simulink library "casper_library_misc"  (R2021a)
settings: Solver=ode45  StartTime=0.0  StopTime=10.0  RelTol=1e-3
libraries: xbsIndex_r4 x168, $bdroot x11, xps_library x6, simulink x4
(part 1 of 3)
settings Model: Creator=mdexter  LastModifiedBy=mcb
settings SolverCC: AlgebraicLoopSolver=TrustRegion
settings DataIOCC: LimitDataPoints=on  SaveFormat=Array  SignalLoggingSaveFormat=ModelDataLogs  ReturnWorkspaceOutputs=off
settings OptimizationCC: BlockReduction=off  BooleanDataType=off  ExpressionDepthLimit=2147483647  LifeSpan=inf
settings DebuggingCC: SaveWithParameterizedLinksMsg=none  UnderspecifiedInitializationDetection=Classic  MergeDetectMultiDrivingBlocksExec=none  SignalResolutionControl=TryResolveAllWithWarning  FcnCallInpInsideContextMsg=warning  AllowSymbolicDim=off  StateNameClashWarn=warning  SFUnexpectedBacktrackingDiag=warning  SFNoUnconditionalDefaultTransitionDiag=warning  SFExecutionAtInitializationDiag=none  SFMachineParentedDataDiag=warning  ArithmeticOperatorsInVariantConditions=warning
settings HardwareCC: ProdBitPerPointer=32  ProdBitPerSizeT=32  ProdBitPerPtrDiffT=32  ProdLargestAtomicFloat=None  ProdIntDivRoundTo=Undefined  ProdEndianess=Unspecified  ProdWordSize=32  ProdHWDeviceType=32-bit Generic  TargetUnknown=on
settings ModelReferenceCC: PropagateSignalLabelsOutOfModel=off
settings SFSimCC: SimUseLocalCustomCode=off  CustomCodeUndefinedFunction=UseInterfaceOnly
settings RTWCC: RTWUseLocalCustomCode=off
settings CodeAppCC: StateflowObjectComments=on
settings GRTTargetCC: TargetLangStandard=C89/C90 (ANSI)  CombineOutputUpdateFcns=off  GRTInterface=on
settings ConfigComp: CovMetricSettings=dw  CovSaveCumulativeToWorkspaceVar=on  CovSaveSingleToWorkspaceVar=on  CovExternalEMLEnable=off

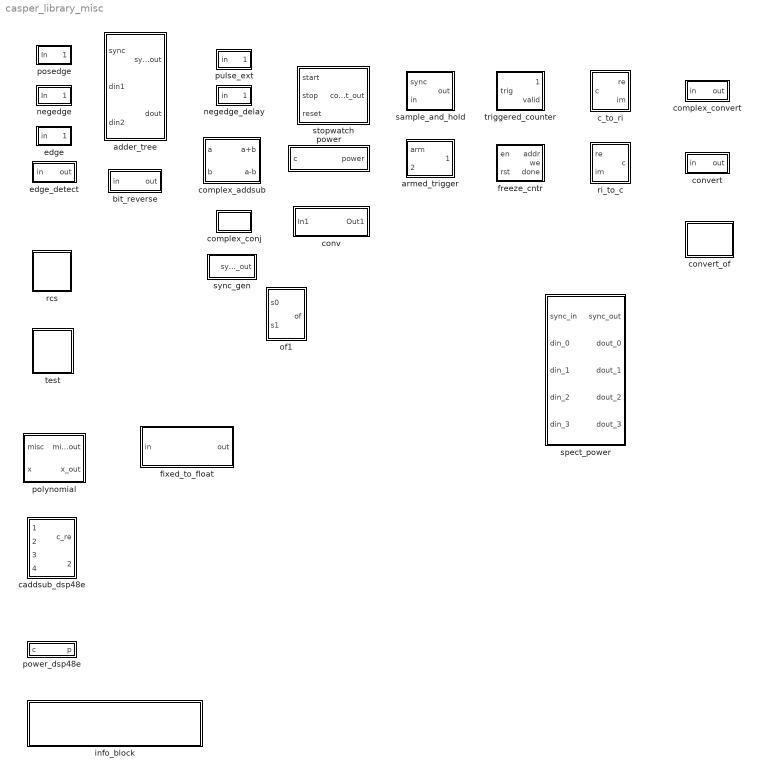
== system casper_library_misc ==
  adder_tree : Subsystem  mask(adder_tree){n_inputs=2, csp_latency=1, adder_imp=Fabric, first_stage_hdl=on, floating_point=off, dvalid_en=off, float_type=single, frac_width=0, exp_width=0}
      mask prompts: n_inputs "Number of Inputs"; csp_latency "Add Latency"; adder_imp "Adder implementation"; first_stage_hdl "Use behavioural HDL for first stage of adders"; floating_point "floating point"; float_type "float type"; frac_width "fraction length"; exp_width "exponent length"
      mask help:
      | Sums all inputs using a tree of adds and delays.
      |
      | Number of inputs: The number of inputs to the block to be summed
      | Add latency: The number of clock cycles to perform one addition (affects timing)..
      | Adder implementation: choice of fabric or DSP48E core, or behavioral HDL
      | Use behavioural HDL for first stage of adders: Causes the first stage of adders to be absorbed into DSP blocks if multipliers precede them (Virtex 5). Overrides Adder implementation
      mask init:
      | adder_tree_init(gcb, ...
      |     'n_inputs', n_inputs, ...
      |     'csp_latency', csp_latency, ...
      |     'adder_imp', adder_imp, ...
      |     'dvalid_en', dvalid_en, ...
      |     'floating_point', floating_point, ...
      |     'float_type', float_type, ...
      |     'exp_width', exp_width, ...
      |     'frac_width', frac_width, ...     
      |     'first_stage_hdl', first_stage_hdl);
      settings: AttributesFormatString=latency 1
      mask Help: eval('xlWeb(''http://casper.berkeley.edu/wiki/Adder_tree'')')
      mask TypeOptions adder_imp: Behavioral | Fabric | DSP48
      mask Callback floating_point:
      | onoff = get_param(gcb, 'floating_point');
      | if strcmp(onoff,'on')
      |     enable_fixpt = 'off';
      |     set_param_state(gcb, 'float_type', 'on')
      | 
      |     f_type = get_param(gcb, 'float_type');
      |     if strcmp(f_type,'custom')
      |         set_param_state(gcb, 'exp_width', 'on')
      |         set_param_state(gcb, 'frac_width', 'on')
      |     else
      |         set_param_state(gcb, 'exp_width', 'off')
      |         set_param_state(gcb, 'frac_width', 'off')
      |     end
      | 
      | 
      | else
      |     enable_fixpt = 'on';
      |     set_param_state(gcb, 'float_type', 'off')
      |     set_param_state(gcb, 'exp_width', 'off')
      |     set_param_state(gcb, 'frac_width', 'off')
      | end
      mask TypeOptions float_type: single | custom
      mask Callback float_type:
      | f_type = get_param(gcb, 'float_type');
      | if strcmp(f_type,'custom')
      |     set_param_state(gcb, 'exp_width', 'on')
      |     set_param_state(gcb, 'frac_width', 'on')
      | else
      |     set_param_state(gcb, 'exp_width', 'off')
      |     set_param_state(gcb, 'frac_width', 'off')
      | end
  armed_trigger : Subsystem  mask(Armed Trigger){}
      mask help: Makes a boolean trigger signal armable.
      mask Help: The trig_out port will go high for one cycle during the first high cycle of trig_in.  Thereafter, trig_out will only go high for one cycle during the first high cycle of trig_in after each rising edge of arm.
  bit_reverse : Subsystem  mask(bit_reverse){n_bits=1}
      mask prompts: n_bits "Number of Bits"
      mask help: Reverses the bit order of the input. Input must be unsigned with binary point at position 0. Costs nothing in hardware.
      mask init:
      | bit_reverse_init(gcb,'n_bits', n_bits);
      settings: AttributesFormatString=1 bits
      mask Help: eval('xlWeb(''http://casper.berkeley.edu/wiki/Bit_reverse'')')
  c_to_ri : Subsystem  mask(c_to_ri){n_bits=8, bin_pt=7}
      mask prompts: n_bits "Bit Width"; bin_pt "Binary Point"
      mask help:
      | Outputs real and imaginary components of a complex input.
      | Useful for simplifying interconnects.
      | See also: Real-Imag to Complex (ri_to_c)
      mask init:
      | annotation=sprintf('%d_%d r/i',n_bits,bin_pt);
      | set_param(gcb,'AttributesFormatString',annotation);
      settings: AttributesFormatString=8_7 r/i
      mask Help: eval('xlWeb(''http://casper.berkeley.edu/wiki/C_to_ri'')')
  caddsub_dsp48e : Subsystem  mask(caddsub_dsp48e){mode=Addition, n_bits_a=18, bin_pt_a=17, n_bits_b=8, bin_pt_b=7, full_precision=on, n_bits_c=19, bin_pt_c=17, quantization=Truncate, overflow=Wrap, cast_latency=0}
      mask prompts: mode "Operation:"; n_bits_a "Bit width 'a':"; bin_pt_a "Binary point 'a':"; n_bits_b "Bit width 'b':"; bin_pt_b "Binary point 'b':"; full_precision "Full precision"; n_bits_c "Bit width out:"; bin_pt_c "Binary point out:"; cast_latency "Cast Latency:"
      mask help:
      | Adds or subtracts two complex numbers using a DSP48E.
      |
      | The two inputs can have different bit widths and binary points, but their sum cannot exceed 24 bits.
      mask init:
      | caddsub_dsp48e_init(gcb, ...
      |     'mode', mode, ...
      |     'n_bits_a', n_bits_a, ...
      |     'bin_pt_a', bin_pt_a, ...
      |     'n_bits_b', n_bits_b, ...
      |     'bin_pt_b', bin_pt_b, ...
      |     'full_precision', full_precision, ...
      |     'n_bits_c', n_bits_c, ...
      |     'bin_pt_c', bin_pt_c, ...
      |     'quantization', quantization, ...
      |     'overflow', overflow, ...
      |     'cast_latency', cast_latency);
      settings: AttributesFormatString=|
      | 18_17 + 8_7 ==> 19_17
      | Mode=Addition
      | Latency=2
      mask TypeOptions mode: Addition | Subtraction
      mask Callback full_precision:
      | thisVariable = 'full_precision';
      | affectedVars = { ...
      |     'n_bits_c', ...
      |     'bin_pt_c', ...
      |     'quantization', ...
      |     'overflow', ...
      |     'cast_latency', ...
      | };
      | 
      | thisBlock = gcb();
      | thisVarState = get_param(thisBlock, thisVariable);
      | maskNames = get_param(thisBlock, 'MaskNames');
      | maskEnables = get_param(thisBlock, 'MaskEnables');
      | 
      | if strcmp(thisVarState, 'on'),
      |     targVarState = 'off';
      | else,
      |     targVarState = 'on';
      | end
      | 
      | for varName = affectedVars
      |     varIndex = find(ismember(maskNames, varName));
      |     maskEnables{varIndex} = targVarState;
      | end
      | 
      | set_param(thisBlock, 'MaskEnables', maskEnables);
      mask TypeOptions quantization: Truncate | Round  (unbiased: +/- Inf) | Round  (unbiased: Even Values)
      mask TypeOptions overflow: Wrap | Saturate | Flag as error
  complex_addsub : Subsystem  mask(complex_addsub){BitWidth=18, add_latency=2}
      mask prompts: BitWidth "Bit Wdith"; add_latency "Add Latency"
      mask help:
      | Adds and subtracts the complex inputs.
      | If a = w + ix, b = y + iz then
      | a+b = (w+y)/2 + i(x-z)/2 and
      | a-b = (x+z)/2 + i(y-w)/2
  complex_conj : Subsystem  mask(complex_conj){n_inputs=0, n_bits=18, bin_pt=17, csp_latency=1, overflow=Wrap, floating_point=on, float_type=single, exp_width=8, frac_width=24}
      mask prompts: n_inputs "number simultaneous inputs"; n_bits "input bitwidth"; bin_pt "input binary point"; csp_latency "latency"; overflow "overflow strategy"; floating_point "floating point"; exp_width "exponent width"; frac_width "fraction width"
      mask help: Finds the complex conjugate of complex inputs.
      mask init:
      | complex_conj_init(gcb, ...
      |     'n_inputs', n_inputs, ...
      |     'n_bits', n_bits, ...
      |     'bin_pt', bin_pt, ...
      |     'floating_point', floating_point, ...
      |     'float_type', float_type, ...
      |     'exp_width', exp_width, ...
      |     'frac_width', frac_width, ...        
      |     'csp_latency', csp_latency, ...
      |     'overflow', overflow);
      mask TypeOptions overflow: Wrap | Saturate | Flag as error
      mask Callback floating_point:
      | onoff = get_param(gcb, 'floating_point');
      | if strcmp(onoff,'on')
      |     enable_fixpt = 'off'
      |     set_param_state(gcb, 'float_type', 'on')
      | 
      |     f_type = get_param(gcb, 'float_type')
      |     if strcmp(f_type,'custom')
      |         set_param_state(gcb, 'exp_width', 'on')
      |         set_param_state(gcb, 'frac_width', 'on')
      |     else
      |         set_param_state(gcb, 'exp_width', 'off')
      |         set_param_state(gcb, 'frac_width', 'off')
      |     end
      | 
      | 
      | else
      |     enable_fixpt = 'on'
      |     set_param_state(gcb, 'float_type', 'off')
      |     set_param_state(gcb, 'exp_width', 'off')
      |     set_param_state(gcb, 'frac_width', 'off')
      | end
      | 
      | set_param_state(gcb, 'n_bits', enable_fixpt)
      | set_param_state(gcb, 'bin_pt', enable_fixpt)
      mask TypeOptions float_type: single | custom
      mask Callback float_type:
      | f_type = get_param(gcb, 'float_type')
      | if strcmp(f_type,'custom')
      |     set_param_state(gcb, 'exp_width', 'on')
      |     set_param_state(gcb, 'frac_width', 'on')
      | else
      |     set_param_state(gcb, 'exp_width', 'off')
      |     set_param_state(gcb, 'frac_width', 'off')
      | end
  complex_convert : Subsystem  mask(complex_convert){n_bits_in=8, bin_pt_in=7, n_bits_out=8, bin_pt_out=7, quantization=Truncate, overflow=Wrap, csp_latency=3}
      mask prompts: n_bits_in "Bit Width In"; bin_pt_in "Binary Point In"; n_bits_out "Bit Width Out"; bin_pt_out "Binary Point Out"; csp_latency "Latency"
      mask help: Convert real and imaginary components of a complex input to the specified bit width and precision.
      mask init:
      | complex_convert_init(gcb, ...
      |     'n_bits_in',n_bits_in,...
      |     'bin_pt_in',bin_pt_in, ...
      |     'n_bits_out',n_bits_out,...
      |     'bin_pt_out',bin_pt_out,...
      |     'quantization',quantization,...
      |     'overflow',overflow,...
      |     'latency',csp_latency);
      settings: AttributesFormatString=|
      | 8_7 ==> 8_7
      | truncate, wrap
      | latency = 3
      mask Help:
      | <pre>
      | Description::
      | 
      | Outputs (complex) converted version of the (complex) input.
      | 
      | Mask Parameters::
      | 
      | Bit Width In (n_bits_in): Specifies the width of the real/imaginary input components.
      | Assumed equal for both components.
      | 
      | Binary Point In (bin_pt_in): Specifies the binary point location in the real/imag input components.
      | Assumed equal for both components.
      | 
      | Bit Width Out (n_bits_out): Specifies the width of the real/imaginary output components.
      | Assumed equal for both components.
      | 
      | Binary Point Out (bin_pt_out): Specifies the binary point location in the real/imag output components.
      | Assumed equal for both components.
      | 
      | Quantization (quantization): Specifies quantization handling.
      | 
      | Overflow (overflow): Specifies overflow handling.
      | 
      | Latency (latency): Specifies the latency of the underlying convert blocks, which is the overall
      | latency of this block as well.
      | </pre>
      mask TypeOptions quantization: Truncate | Round  (unbiased: +/- Inf) | Round  (unbiased: Even Values)
      mask TypeOptions overflow: Wrap | Saturate | Error
  conv : Subsystem
      mask help:
      | Converts an (8-bit) unsigned number to 2's complement.
      | This block should eventually be able to handle arbitrary
      | width inputs.
  convert : Subsystem  mask(convert){bin_pt_in=7, n_bits_out=4, bin_pt_out=3, quantization=Truncate, overflow=Wrap, csp_latency=4, implementation=0}
      mask prompts: bin_pt_in "Binary Point In"; n_bits_out "Bit Width Out"; bin_pt_out "Binary Point Out"; csp_latency "Latency"; implementation "Implementation (0=Fabric Core, 1=DSP Core, 2=Behavioural)"
      mask help:
      | Convert input value to the specified bit width and precision.
      |
      | Does not support upscaling number of fractional bits (eg 8_5 to 8_4 is ok, but not 8_4 to 8_5).
      mask init:
      | convert_init(gcb, ...
      |     'bin_pt_in',bin_pt_in, ...
      |     'n_bits_out',n_bits_out,...
      |     'bin_pt_out',bin_pt_out, ...
      |     'quantization',quantization,...
      |     'overflow',overflow,...
      |     'csp_latency',csp_latency,...
      |     'implementation', implementation);
      settings: AttributesFormatString=|
      | N_7 ==> 4_3
      | truncate, wrap
      | latency = 4
      mask Help:
      | <pre>
      | Description::
      | 
      | Outputs converted version of the input.
      | 
      | Mask Parameters::
      | 
      | Binary Point In (bin_pt_in): Specifies the binary point location in the input.
      | 
      | Bit Width Out (n_bits_out): Specifies the width of the output.
      | 
      | Binary Point Out (bin_pt_out): Specifies the binary point location in the output.
      | 
      | Quantization (quantization): Specifies quantization handling.
      | 
      | Overflow (overflow): Specifies overflow handling.
      | 
      | Latency (latency): Specifies the latency of the underlying adder block, which is the overall
      | latency of this block as well.
      | </pre>
      mask TypeOptions quantization: Truncate | Round  (unbiased: +/- Inf) | Round  (unbiased: Even Values) | Round  (unbiased: Zero) | Round  (unbiased: Odd Values) | Round  (biased: Up) | Round  (biased: Down)
      mask TypeOptions overflow: Wrap | Saturate | Error
  convert_of : Subsystem  mask(convert_of){bit_width_i=0, binary_point_i=2, bit_width_o=8, binary_point_o=7, csp_latency=2, overflow=Wrap, quantization=Truncate}
      mask prompts: bit_width_i "Bit Width In"; binary_point_i "Binary Point In"; bit_width_o "Bit Width Out"; binary_point_o "Binary Point Out"; csp_latency "Latency"; overflow "Overflow Behaviour"; quantization "Quantization Behaviour"
      mask help:
      | Converts from one 2's complement bit-width
      | and/or binary point position to another.
      | Includes underflow/overflow indicator.
      mask init:
      | convert_of_init(gcb, ...
      |     'bit_width_i', bit_width_i, ...
      |     'binary_point_i', binary_point_i, ...
      |     'bit_width_o', bit_width_o, ...
      |     'binary_point_o', binary_point_o, ...
      |     'latency',csp_latency, ...
      |     'overflow', overflow, ...
      |     'quantization', quantization);
      mask TypeOptions overflow: Wrap | Saturate | Error
      mask TypeOptions quantization: Truncate | Round  (unbiased: +/- Inf) | Round  (unbiased: even values)
  edge : Subsystem  mask(edge){}
      mask help: Outputs true if a boolean input signal is not equal to its value last clock.
      mask init:
      | deprecation_warning('the edge block is to be removed from the casper library, please use the edge_detect block instead', 'edge');
      settings: CopyFcn=deprecation_warning('the edge block is to be removed from the casper library, please use the edge_detect block instead','edge')
      mask Help: eval('xlWeb(''http://casper.berkeley.edu/wiki/Edge'')')
  edge_detect : Subsystem  mask(edge_detect){edge=Rising, polarity=Active High, x_in=[0 0.08 0.08 0.16 0.16 0.24 0.24 0.32 0.32 0.4], y_in=[-1 -1  1  1  1  1  1  1  1  1], x_out=[0.6 0.68 0.68 0.76 0.76 0.84 0.84 0.92 0.92 1], y_out=[-1 -1  1  1 -1 -1 -1 -1 -1 -1]}
      mask prompts: edge "Edge Type"; polarity "Output Polarity"; x_in "Input X Positions"; y_in "Input Y Positions"; x_out "Output X Positions"; y_out "Output Y Positions"
      mask help: Output is active for one-cycle after each edge of the specified type (i.e. rising, falling or both).
      mask init:
      | edge_detect_init(gcb,...
      |     'edge',edge,...
      |     'polarity',polarity,...
      |     'x_in',x_in,...
      |     'x_out',x_out,...
      |     'y_in',y_in,...
      |     'y_out',y_out);
      | 
      | x_in_num=str2num(getfield(getfield(get_param(gcb,'UserData'),'parameters'),'x_in'));
      | x_out_num=str2num(getfield(getfield(get_param(gcb,'UserData'),'parameters'),'x_out'));
      | y_in_num=str2num(getfield(getfield(get_param(gcb,'UserData'),'parameters'),'y_in'));
      | y_out_num=str2num(getfield(getfield(get_param(gcb,'UserData'),'parameters'),'y_out'));
      settings: AttributesFormatString=|
      | rising edges
      | active high
      mask Help: Output is active for one-cycle after each edge of the specified type (i.e. rising, falling, or both).  Latency is zero.
      mask TypeOptions edge: Rising | Falling | Both
      mask TypeOptions polarity: Active High | Active Low
      mask Display:
      | plot(x_in_num,0.5+y_in_num*0.2);
      | plot(x_out_num,0.5+y_out_num*0.2);
  fixed_to_float : Subsystem  mask(fixed_to_float){float_type=single, n_bits_in=18, bin_pt=17, num_vec=1, csp_latency=0}
      mask prompts: float_type "float type"; n_bits_in "input word length"; bin_pt "input binary point"; num_vec "number vectors in bus"; csp_latency "Latency"
      mask help: Convert fixed point vector (or bus of) to flaoting point
      mask TypeOptions float_type: single | custom
  freeze_cntr : Subsystem  mask(freeze_cntr){CounterBits=5}
      mask prompts: CounterBits "Counter Length (2^?)"
      mask help:
      | A freeze counter is an enabled counter which holds its final value (regardless of enables)
      | until it is reset.
      mask Help: eval('xlWeb(''http://casper.berkeley.edu/wiki/Freeze_cntr'')')
  info_block : Subsystem  Tag=casper:info  mask(comment_block){info=Any information about this system\nthat should be readable from software.\nSee documentation.}
      mask help:
      | Any comment made using this block will be parsed by the toolflow and stored in the bitstream, accessible by software.
      | It's an unevaluated string, and some characters make Matlab unhappy, so the user must define/find a data transport format if that is the intended purpose.
      settings: MoveFcn=pos = get_param(gcb, 'Position'); height = pos(4)-pos(2); txt = get_param(gcb, 'info'); set_param(gcb,'MaskValueString',txt);
      mask Display:
      | pos = get_param(gcb, 'Position');
      | height = pos(4)-pos(2);
      | txt = get_param(gcb, 'info');
      | text(10,height/2,txt);
  negedge : Subsystem  Tag=Rising Edge Detector  mask(negedge){}
      mask help: Outputs true if a boolean input signal is currently false, but was true last clock.
      mask init:
      | deprecation_warning('the negedge block is to be removed from the casper library, please use the edge_detect block instead', 'negedge');
      settings: CopyFcn=deprecation_warning('the negedge block is to be removed from the casper library, please use the edge_detect block instead','negedge')
      mask Help: eval('xlWeb(''http://casper.berkeley.edu/wiki/Negedge'')')
  negedge_delay : Subsystem  mask(negedge_delay){pulse_len=5}
      mask prompts: pulse_len "Length of Pulse"
      mask help:
      | Extends a boolean signal to be high for the specified number of clocks after
      | the last high input (negative edge).
      |
      | Minimum length is 3.
      mask init:
      | bits = ceil(log2(pulse_len+1));
      | 
      | if pulse_len < 3,
      |     errordlg('Minimum length is 3.');
      | end
  of1 : Subsystem  mask(of){bit_num=0, n_adc_bits=8}
      mask prompts: bit_num "Bit index of overflow detection bus:"; n_adc_bits "Number of bits in ADC"
      mask help: 1-cycle overflow detector for an n-bit ADC outputs (simulation only)
  polynomial : Subsystem  mask(polynomial){n_polys=0, degree=0, mult_latency=2, bits_out=18, bin_pt_out=17, conv_latency=2, quantization=Truncate, overflow=Wrap, bits_in=8, bin_pt_in=0}
      mask prompts: n_polys "Number of polynomials"; degree "Degree of polynomial"; mult_latency "Multiplier latency"; bits_out "Output number of bits"; bin_pt_out "Output binary point"; conv_latency "Convert latency"; quantization "Quantization behaviour"; overflow "Overflow behaviour"; bits_in "Bits in"; bin_pt_in "Binary point in"
      mask init:
      | polynomial_init(gcb, ...
      |     'n_polys', n_polys, ...
      |     'degree', degree, ...
      |     'mult_latency', mult_latency, ...
      |     'bits_out', bits_out, ...
      |     'bin_pt_out', bin_pt_out, ...
      |     'conv_latency', conv_latency, ...
      |     'quantization', quantization, ...
      |     'overflow', overflow, ...
      |     'bits_in', bits_in, ...
      |     'bin_pt_in', bin_pt_in);
      mask TypeOptions quantization: Truncate | Round  (unbiased: +/- Inf) | Round  (unbiased: even values)
      mask TypeOptions overflow: Wrap | Saturate | Error
  posedge : Subsystem  Tag=Rising Edge Detector  mask(posedge){}
      mask help: Outputs true if a boolean input signal is true this clock and was false last clock.
      mask init:
      | deprecation_warning('the posedge block is to be removed from the casper library, please use the edge_detect block instead', 'posedge');
      settings: CopyFcn=deprecation_warning('the posedge block is to be removed from the casper library, please use the edge_detect block instead','posedge')
      mask Help: eval('xlWeb(''http://casper.berkeley.edu/wiki/Posedge'')')
  power : Subsystem  mask(power){BitWidth=18, add_latency=2, mult_latency=3}
      mask prompts: BitWidth "Bit Width"; add_latency "Add Latency"; mult_latency "Mult Latency"
      mask help: Squares real and imaginary components of complex input and adds them.
      mask Help: eval('xlWeb(''http://casper.berkeley.edu/wiki/Power'')')
      mask Display:
      | port_label('input', 1, 'c');
      | port_label('output', 1, 'power');
      | disp(['Z^-', num2str(mult_latency+add_latency)]);
  power_dsp48e : Subsystem  mask(power_dsp48e){bitwidth=18}
      mask prompts: bitwidth "Input bit width:"
      mask help: Computes the power of a complex number using 2 DSP48Es.
      mask Display:
      | port_label('input', 1, 'c');
      | port_label('output', 1, 'p');
      | disp(['Z^-', num2str(4)]);
  pulse_ext : Subsystem  mask(pulse_ext){pulse_len=5}
      mask prompts: pulse_len "Length of Pulse"
      mask help:
      | Extends a boolean signal to be high for the specified number of clocks after
      | the last high input.
      mask init:
      | bits = ceil(log2(pulse_len+1));
      mask Help: eval('xlWeb(''http://casper.berkeley.edu/wiki/Pulse_ext'')')
  rcs : Subsystem  mask(rcs){app_src=timestamp, lib_src=timestamp, user_val=0}
      mask prompts: app_src "Application revision info to capture"; lib_src "CASPER libraries revision info to capture"; user_val "User specified value"
      mask help:
      | Embeds revision control information for the user design and libraries.
      | On failure to locate specified revision information, falls back to
      | timestamps (current time for libraries).
      | A user specified value is also stored.
      mask init:
      | rcs_init(gcb, ...
      |     'app_src', app_src, ...
      |     'lib_src', lib_src);
      mask TypeOptions app_src: timestamp | git | svn
      mask TypeOptions lib_src: timestamp | git | svn
  ri_to_c : Subsystem  mask(ri_to_c){}
      mask help:
      | Concatenates real and imaginary inputs into a complex output.
      | Useful for simplifying interconnects.
      | See also: Complex to Real-Imag (c_to_ri)
      mask Help: eval('xlWeb(''http://casper.berkeley.edu/wiki/Ri_to_c'')')
  sample_and_hold : Subsystem  mask(sample_and_hold){period=1024}
      mask prompts: period "Sample period (clocks)"
      mask help: This block will sample an input signal at a user specified rate and hold the value on the output.
  spect_power : Subsystem  mask{bitwidth=18, add_latency=2, mult_latency=3, mode=dsp48e, n_inputs=4}
      mask prompts: bitwidth "Bit Width"; add_latency "Adder Latency"; mult_latency "Mult Latency"; n_inputs "Number of Inputs"
      mask init:
      | config.source = str2func('spect_power');
      | config.depend = {'spect_power.m'};
      | config.toplevel = gcb;
      | xBlock(config, {bitwidth, add_latency, mult_latency, mode, n_inputs});
      mask TypeOptions mode: behavioral | dsp48e
  stopwatch : Subsystem  mask(stopwatch){}
      mask help: Counts the number of clocks between a start and stop pulse.
      mask Help: eval('xlWeb(''http://casper.berkeley.edu/wiki/Stopwatch'')')
  sync_gen : Subsystem  mask(sync_gen){sim_acc_len=7, fft_size=256, fft_simult_inputs=8, pfb_fir_taps=4, reorder_vec=getfield( getfield( get_param( gcb,'UserData' ), 'parameters'),'reorder_vec'), scale=1}
      mask prompts: sim_acc_len "Simulation Accumulation Length"; fft_size "FFT Size"; fft_simult_inputs "Simultaneous Inputs (FFT)"; pfb_fir_taps "Taps in pfb_fir (use 1 if no pfb_fir)"; reorder_vec "Reorder Orders (e.g. [2 2 2])"
      mask help:
      | This block computes the sync period based on system parameters as
      | described in Casper memo.  Detailed descritions of the block's
      | variables can be found in the 'Block Documentation' section of
      | the CASPER wiki.
      mask init:
      | sync_gen_init(gcb, ...
      |     'sim_acc_len', sim_acc_len, ...
      |     'fft_size', fft_size, ...
      |     'fft_simult_inputs', fft_simult_inputs,...
      |     'pfb_fir_taps', pfb_fir_taps, ...
      |     'reorder_vec', reorder_vec, ...
      |     'scale', scale);
      settings: AttributesFormatString=sim_sync_period=8960
      mask Help:
      | SyncPeriod=LCM(reorder_vec)*(acc_num)*(pfb_fir_len)*(fft_size/fft_simult_inputs)
      | 
      | See CASPER sync pulse memo for more details.
  test : Subsystem  mask(test){tests_location=/opt/casper_git_devel/casper_library/Tests, tests_file=tester_input.txt, test_type=section from block, subsection=Downconverter, block=lo_osc, stop_first_fail=on}
      mask prompts: tests_location "Location of unit tests"; tests_file "Name of test file"; test_type "Test type:"; subsection "Library subsection:"; block "Library block"; stop_first_fail "Stop testing on first failure"
      mask help: Interface to test infrastruture
      mask init:
      | test_init( gcb, ...
      |     'tests_location', tests_location, ...
      |     'tests_file', tests_file, ...
      |     'test_type', test_type, ...
      |     'subsection', subsection, ...
      |     'block', block, ...
      |     'stop_first_fail', stop_first_fail);
      mask Callback tests_file:
      | %ideally, generate sections and blocks
      | %from tests_location and test_file
      mask TypeOptions test_type: all | section | section from block | unit
  triggered_counter : Subsystem  mask{len=8}
      mask prompts: len "Run Length"

== system casper_library_misc/adder_tree ==
  sync : Inport
  din1 : Inport  Port=2
  din2 : Inport  Port=3
  addr1 : xbsIndex_r4/AddSub  mode=Addition  use_carryin=off  use_carryout=off  en=off  latency=1  precision=Full  arith_type=Unsigned  n_bits=16  bin_pt=14  quantization=Truncate  overflow=Wrap  use_behavioral_HDL=on  hw_selection=Fabric  pipelined=on  use_rpm=on  dbl_ovrd=off  block_type=addsub
  sync_delay : xbsIndex_r4/Delay  rst=off  infoeditControl=Selection of Reset will increase slice count due to use of real FFs and instead of SRLs  en=off  latency=1  reg_retiming=on  dbl_ovrd=off  block_type=delay
      settings: block_version=11.4
  sync_out : Outport  VectorParamsAs1DForOutWhenUnconnected=off
  dout : Outport  Port=2  VectorParamsAs1DForOutWhenUnconnected=off
  wires:
  sync/1 -> sync_delay/1
  sync_delay/1 -> sync_out/1
  din1/1 -> addr1/1
  din2/1 -> addr1/2
  addr1/1 -> dout/1

== system casper_library_misc/armed_trigger ==
  arm : Inport
  trig_in : Inport  Port=2
  Constant2 : xbsIndex_r4/Constant  const=0  gui_display_data_type=Fixed-point  arith_type=Boolean  n_bits=1  bin_pt=0  preci_type=Single  exp_width=8  frac_width=24  explicit_period=off  period=1  equ=P=C  opselect=C  inp2=PCIN>>17  opr=+  inp1=P  carry=CIN  dbl_ovrd=off  block_type=constant
  Logical : xbsIndex_r4/Logical  logical_function=AND  inputs=2  en=off  latency=0  precision=Full  arith_type=Unsigned  n_bits=8  bin_pt=2  align_bp=on  dbl_ovrd=off  block_type=logical
      settings: xl_area=[0, 0, 0, 0, 0, 0, 0]
  armed : xbsIndex_r4/Register  init=1  rst=on  en=on  dbl_ovrd=off  block_type=register
      settings: AttributesFormatString=init=%<init>  xl_area=[0, 0, 0, 0, 0, 0, 0]
  edge_detect : Subsystem  mask(edge_detect){edge=Rising, polarity=Active High, xin=floor([0.5:0.5:5])*0.08, yin={[-1,-1,1,1,1,1,1,1,1,1],[1,1,-1,-1,-1,-1,-1,-1,-1,-1],[-1,-1,1,1,1,1,-1,-1,-1,-1]}, xout=1-floor([5:-0.5:0.5])*0.08, yout={[-1,-1,1,1,-1,-1,-1,-1,-1,-1],[-1,-1,1,1,-1,-1,-1,-1,-1,-1],[-1,-1,1,1,-1,-1,1,1,-1,-1]}}
      mask prompts: edge "Edge Type"; polarity "Output Polarity"; xin "Input X Positions"; yin "Input Y Positions"; xout "Output X Positions"; yout "Output Y Positions"
      mask help: Output is active for one-cycle after each edge of the specified type (i.e. rising, falling or both).
      mask init:
      | %edge_detect_init(gcb,edge,polarity);
      settings: AttributesFormatString=|
      | rising edges
      | active high
      mask Help: Output is active for one-cycle after each edge of the specified type (i.e. rising, falling, or both).  Latency is zero.
      mask TypeOptions edge: Rising | Falling | Both
      mask TypeOptions polarity: Active High | Active Low
      mask Display:
      | plot(xin,0.5+yin{edge}*0.2)
      | plot(xout,0.5+yout{edge}*0.2*(3-2*polarity))
  trig_out : Outport  VectorParamsAs1DForOutWhenUnconnected=off
  wires:
  Constant2/1 -> armed/1
  edge_detect/1(out) -> armed/2
  armed/1 -> Logical/1
  Logical/1 -> armed/3, trig_out/1
  arm/1 -> edge_detect/1(in)
  trig_in/1 -> Logical/2

== system casper_library_misc/bit_reverse ==
  in : Inport
  out : Outport  VectorParamsAs1DForOutWhenUnconnected=off
  wires:
  in/1 -> out/1

== system casper_library_misc/c_to_ri ==
  c : Inport
  force_im : xbsIndex_r4/Reinterpret  force_arith_type=on  arith_type="Signed  (2's comp)"  force_bin_pt=on  bin_pt=bin_pt  block_type=reinterpret
      settings: infoedit="Changes signal type without altering the binary representation.   You can changed the signal between signed and unsigned, and relocate the binary point.<P><P>Hardware notes: In hardware this block costs nothing.<P><P>Example:  Suppose the input is 6 bits wide, signed, with 2 fractional bits, and the output is forced to unsigned with 0 fractional bits.  Then an input of -2.0 (1110.00 in binary 2's complement) becomes an output of 56 (111000 in binary)."  block_version=9.1.01
  force_re : xbsIndex_r4/Reinterpret  force_arith_type=on  arith_type="Signed  (2's comp)"  force_bin_pt=on  bin_pt=bin_pt  block_type=reinterpret
      settings: infoedit="Changes signal type without altering the binary representation.   You can changed the signal between signed and unsigned, and relocate the binary point.<P><P>Hardware notes: In hardware this block costs nothing.<P><P>Example:  Suppose the input is 6 bits wide, signed, with 2 fractional bits, and the output is forced to unsigned with 0 fractional bits.  Then an input of -2.0 (1110.00 in binary 2's complement) becomes an output of 56 (111000 in binary)."  block_version=9.1.01
  slice_im : xbsIndex_r4/Slice  nbits=n_bits  boolean_output=off  mode=Lower Bit Location + Width  bit1=0  base1=MSB of Input  bit0=0  base0=LSB of Input  dbl_ovrd=off  block_type=slice
      settings: infoedit="Extracts a given range of bits from each input sample and presents it at the output.  The output type is ordinarily unsigned with binary point at zero, but can be Boolean when the slice is one bit wide.<P><P>Hardware notes: In hardware this block costs nothing."  block_version=9.1.01
  slice_re : xbsIndex_r4/Slice  nbits=n_bits  boolean_output=off  mode=Upper Bit Location + Width  bit1=0  base1=MSB of Input  bit0=0  base0=LSB of Input  dbl_ovrd=off  block_type=slice
      settings: infoedit="Extracts a given range of bits from each input sample and presents it at the output.  The output type is ordinarily unsigned with binary point at zero, but can be Boolean when the slice is one bit wide.<P><P>Hardware notes: In hardware this block costs nothing."  block_version=9.1.01
  re : Outport  VectorParamsAs1DForOutWhenUnconnected=off
  im : Outport  Port=2  VectorParamsAs1DForOutWhenUnconnected=off
  wires:
  c/1 -> slice_im/1, slice_re/1
  force_im/1 -> im/1
  force_re/1 -> re/1
  slice_im/1 -> force_im/1
  slice_re/1 -> force_re/1

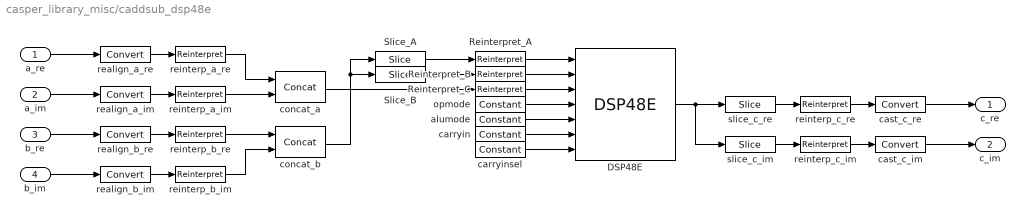
== system casper_library_misc/caddsub_dsp48e ==
  a_re : Inport
  a_im : Inport  Port=2
  b_re : Inport  Port=3
  b_im : Inport  Port=4
  DSP48E : xbsIndex_r4/DSP48E  use_a=Direct from A Port  use_b=Direct from B Port  reset_preg=off  pattern_from_creg=off  pattern='000000000000'  mask_from_creg=off  pattern_mask='3FFFFFFFFFFF'  sel_rounding_mask=Select mask  use_op=off  use_creg=on  rst_all=off  en_all=off  use_pcin=off  use_carrycascin=off  use_multsignin=off  use_carryout=off  use_patterndetect=off  use_patternbdetect=off  use_overflow=off  use_underflow=off  use_acout=off  use_bcout=off  use_pcout=off  use_multsignout=off  use_carrycascout=off  pipeline_a=1  pipeline_b=1  pipeline_acout=1  pipeline_bcout=1  pipeline_c=on  pipeline_p=on  pipeline_mult=on  pipeline_opmode=on  pipeline_alumode=on  pipeline_carryin=on  pipeline_carryinsel=on  rst_a=off  rst_b=off  rst_c=off  rst_mult=off  rst_p=off  rst_carry_in=off  rst_alumode=off  rst_ctrl=off  en_a1=off  en_a2=off  en_b1=off  en_b2=off  en_c=off  en_mult=off  en_p=off  en_carry_in=off  en_alumode=off  en_multcarryin=off  en_ctrl=off  use_synth_model=off  addsub_mode=TWO24  xl_useadderonly=off  block_type=dsp48e
      settings: block_version=10.1.3
  Reinterpret_A : xbsIndex_r4/Reinterpret  force_arith_type=on  arith_type="Signed  (2's comp)"  force_bin_pt=on  bin_pt=0  block_type=reinterpret
      settings: infoedit="Changes signal type without altering the binary representation.   You can changed the signal between signed and unsigned, and relocate the binary point.<br><br>Hardware notes: In hardware this block costs nothing.<br><br>Example:  Suppose the input is 6 bits wide, signed, with 2 fractional bits, and the output is forced to unsigned with 0 fractional bits.  Then an input of -2.0 (1110.00 in binary 2's complement) becomes an output of 56 (111000 in binary)."  block_version=10.1.3
  Reinterpret_B : xbsIndex_r4/Reinterpret  force_arith_type=on  arith_type="Signed  (2's comp)"  force_bin_pt=on  bin_pt=0  block_type=reinterpret
      settings: infoedit="Changes signal type without altering the binary representation.   You can changed the signal between signed and unsigned, and relocate the binary point.<br><br>Hardware notes: In hardware this block costs nothing.<br><br>Example:  Suppose the input is 6 bits wide, signed, with 2 fractional bits, and the output is forced to unsigned with 0 fractional bits.  Then an input of -2.0 (1110.00 in binary 2's complement) becomes an output of 56 (111000 in binary)."  block_version=10.1.3
  Reinterpret_C : xbsIndex_r4/Reinterpret  force_arith_type=on  arith_type="Signed  (2's comp)"  force_bin_pt=on  bin_pt=0  block_type=reinterpret
      settings: infoedit="Changes signal type without altering the binary representation.   You can changed the signal between signed and unsigned, and relocate the binary point.<br><br>Hardware notes: In hardware this block costs nothing.<br><br>Example:  Suppose the input is 6 bits wide, signed, with 2 fractional bits, and the output is forced to unsigned with 0 fractional bits.  Then an input of -2.0 (1110.00 in binary 2's complement) becomes an output of 56 (111000 in binary)."  block_version=10.1.3
  Slice_A : xbsIndex_r4/Slice  nbits=30  boolean_output=off  mode=Upper Bit Location + Width  bit1=0  base1=MSB of Input  bit0=0  base0=LSB of Input  dbl_ovrd=off  block_type=slice
  Slice_B : xbsIndex_r4/Slice  nbits=18  boolean_output=off  mode=Lower Bit Location + Width  bit1=0  base1=MSB of Input  bit0=0  base0=LSB of Input  dbl_ovrd=off  block_type=slice
  alumode : xbsIndex_r4/Constant  const=0  gui_display_data_type=Fixed-point  arith_type=Unsigned  n_bits=4  bin_pt=0  preci_type=Single  exp_width=8  frac_width=24  explicit_period=off  period=1  equ=P=C  opselect=C  inp2=PCIN>>17  opr=+  inp1=P  carry=CIN  dbl_ovrd=off  block_type=constant
  carryin : xbsIndex_r4/Constant  const=0  gui_display_data_type=Fixed-point  arith_type=Unsigned  n_bits=1  bin_pt=0  preci_type=Single  exp_width=8  frac_width=24  explicit_period=off  period=1  equ=P=C  opselect=C  inp2=PCIN>>17  opr=+  inp1=P  carry=CIN  dbl_ovrd=off  block_type=constant
  carryinsel : xbsIndex_r4/Constant  const=0  gui_display_data_type=Fixed-point  arith_type=Unsigned  n_bits=3  bin_pt=0  preci_type=Single  exp_width=8  frac_width=24  explicit_period=off  period=1  equ=P=C  opselect=C  inp2=PCIN>>17  opr=+  inp1=P  carry=CIN  dbl_ovrd=off  block_type=constant
  cast_c_im : xbsIndex_r4/Convert  gui_display_data_type=Fixed-point  arith_type="Signed  (2's comp)"  n_bits=19  bin_pt=17  float_type=Single  exp_bits=8  fraction_bits=24  quantization=Truncate  overflow=Wrap  en=off  latency=0  pipeline=on  dbl_ovrd=off  block_type=convert
      settings: block_version=10.1.3
  cast_c_re : xbsIndex_r4/Convert  gui_display_data_type=Fixed-point  arith_type="Signed  (2's comp)"  n_bits=19  bin_pt=17  float_type=Single  exp_bits=8  fraction_bits=24  quantization=Truncate  overflow=Wrap  en=off  latency=0  pipeline=on  dbl_ovrd=off  block_type=convert
      settings: block_version=10.1.3
  concat_a : xbsIndex_r4/Concat  num_inputs=2  dbl_ovrd=off  block_type=concat
  concat_b : xbsIndex_r4/Concat  num_inputs=2  dbl_ovrd=off  block_type=concat
  opmode : xbsIndex_r4/Constant  const=51  gui_display_data_type=Fixed-point  arith_type=Unsigned  n_bits=7  bin_pt=0  preci_type=Single  exp_width=8  frac_width=24  explicit_period=off  period=1  equ=P=C  opselect=C  inp2=PCIN>>17  opr=+  inp1=P  carry=CIN  dbl_ovrd=off  block_type=constant
  realign_a_im : xbsIndex_r4/Convert  gui_display_data_type=Fixed-point  arith_type="Signed  (2's comp)"  n_bits=24  bin_pt=21  float_type=Single  exp_bits=8  fraction_bits=24  quantization=Truncate  overflow=Wrap  en=off  latency=0  pipeline=on  dbl_ovrd=off  block_type=convert
      settings: block_version=10.1.3
  realign_a_re : xbsIndex_r4/Convert  gui_display_data_type=Fixed-point  arith_type="Signed  (2's comp)"  n_bits=24  bin_pt=21  float_type=Single  exp_bits=8  fraction_bits=24  quantization=Truncate  overflow=Wrap  en=off  latency=0  pipeline=on  dbl_ovrd=off  block_type=convert
      settings: block_version=10.1.3
  realign_b_im : xbsIndex_r4/Convert  gui_display_data_type=Fixed-point  arith_type="Signed  (2's comp)"  n_bits=24  bin_pt=21  float_type=Single  exp_bits=8  fraction_bits=24  quantization=Truncate  overflow=Wrap  en=off  latency=0  pipeline=on  dbl_ovrd=off  block_type=convert
      settings: block_version=10.1.3
  realign_b_re : xbsIndex_r4/Convert  gui_display_data_type=Fixed-point  arith_type="Signed  (2's comp)"  n_bits=24  bin_pt=21  float_type=Single  exp_bits=8  fraction_bits=24  quantization=Truncate  overflow=Wrap  en=off  latency=0  pipeline=on  dbl_ovrd=off  block_type=convert
      settings: block_version=10.1.3
  reinterp_a_im : xbsIndex_r4/Reinterpret  force_arith_type=on  arith_type=Unsigned  force_bin_pt=on  bin_pt=0  block_type=reinterpret
      settings: infoedit="Changes signal type without altering the binary representation.   You can changed the signal between signed and unsigned, and relocate the binary point.<br><br>Hardware notes: In hardware this block costs nothing.<br><br>Example:  Suppose the input is 6 bits wide, signed, with 2 fractional bits, and the output is forced to unsigned with 0 fractional bits.  Then an input of -2.0 (1110.00 in binary 2's complement) becomes an output of 56 (111000 in binary)."  block_version=10.1.3
  reinterp_a_re : xbsIndex_r4/Reinterpret  force_arith_type=on  arith_type=Unsigned  force_bin_pt=on  bin_pt=0  block_type=reinterpret
      settings: infoedit="Changes signal type without altering the binary representation.   You can changed the signal between signed and unsigned, and relocate the binary point.<br><br>Hardware notes: In hardware this block costs nothing.<br><br>Example:  Suppose the input is 6 bits wide, signed, with 2 fractional bits, and the output is forced to unsigned with 0 fractional bits.  Then an input of -2.0 (1110.00 in binary 2's complement) becomes an output of 56 (111000 in binary)."  block_version=10.1.3
  reinterp_b_im : xbsIndex_r4/Reinterpret  force_arith_type=on  arith_type=Unsigned  force_bin_pt=on  bin_pt=0  block_type=reinterpret
      settings: infoedit="Changes signal type without altering the binary representation.   You can changed the signal between signed and unsigned, and relocate the binary point.<br><br>Hardware notes: In hardware this block costs nothing.<br><br>Example:  Suppose the input is 6 bits wide, signed, with 2 fractional bits, and the output is forced to unsigned with 0 fractional bits.  Then an input of -2.0 (1110.00 in binary 2's complement) becomes an output of 56 (111000 in binary)."  block_version=10.1.3
  reinterp_b_re : xbsIndex_r4/Reinterpret  force_arith_type=on  arith_type=Unsigned  force_bin_pt=on  bin_pt=0  block_type=reinterpret
      settings: infoedit="Changes signal type without altering the binary representation.   You can changed the signal between signed and unsigned, and relocate the binary point.<br><br>Hardware notes: In hardware this block costs nothing.<br><br>Example:  Suppose the input is 6 bits wide, signed, with 2 fractional bits, and the output is forced to unsigned with 0 fractional bits.  Then an input of -2.0 (1110.00 in binary 2's complement) becomes an output of 56 (111000 in binary)."  block_version=10.1.3
  reinterp_c_im : xbsIndex_r4/Reinterpret  force_arith_type=on  arith_type="Signed  (2's comp)"  force_bin_pt=on  bin_pt=21  block_type=reinterpret
      settings: infoedit="Changes signal type without altering the binary representation.   You can changed the signal between signed and unsigned, and relocate the binary point.<br><br>Hardware notes: In hardware this block costs nothing.<br><br>Example:  Suppose the input is 6 bits wide, signed, with 2 fractional bits, and the output is forced to unsigned with 0 fractional bits.  Then an input of -2.0 (1110.00 in binary 2's complement) becomes an output of 56 (111000 in binary)."  block_version=10.1.3
  reinterp_c_re : xbsIndex_r4/Reinterpret  force_arith_type=on  arith_type="Signed  (2's comp)"  force_bin_pt=on  bin_pt=21  block_type=reinterpret
      settings: infoedit="Changes signal type without altering the binary representation.   You can changed the signal between signed and unsigned, and relocate the binary point.<br><br>Hardware notes: In hardware this block costs nothing.<br><br>Example:  Suppose the input is 6 bits wide, signed, with 2 fractional bits, and the output is forced to unsigned with 0 fractional bits.  Then an input of -2.0 (1110.00 in binary 2's complement) becomes an output of 56 (111000 in binary)."  block_version=10.1.3
  slice_c_im : xbsIndex_r4/Slice  nbits=24  boolean_output=off  mode=Lower Bit Location + Width  bit1=0  base1=MSB of Input  bit0=0  base0=LSB of Input  dbl_ovrd=off  block_type=slice
  slice_c_re : xbsIndex_r4/Slice  nbits=24  boolean_output=off  mode=Lower Bit Location + Width  bit1=0  base1=MSB of Input  bit0=24  base0=LSB of Input  dbl_ovrd=off  block_type=slice
  c_re : Outport  VectorParamsAs1DForOutWhenUnconnected=off
  c_im : Outport  Port=2  VectorParamsAs1DForOutWhenUnconnected=off
  wires:
  cast_c_im/1 -> c_im/1
  cast_c_re/1 -> c_re/1
  reinterp_a_re/1 -> concat_a/1
  reinterp_b_im/1 -> concat_b/2
  reinterp_b_re/1 -> concat_b/1
  reinterp_a_im/1 -> concat_a/2
  concat_b/1 -> Slice_B/1, Slice_A/1
  Reinterpret_C/1 -> DSP48E/3
  reinterp_c_im/1 -> cast_c_im/1
  reinterp_c_re/1 -> cast_c_re/1
  slice_c_im/1 -> reinterp_c_im/1
  slice_c_re/1 -> reinterp_c_re/1
  DSP48E/1 -> slice_c_im/1, slice_c_re/1
  Slice_A/1 -> Reinterpret_A/1
  Slice_B/1 -> Reinterpret_B/1
  concat_a/1 -> Reinterpret_C/1
  b_im/1 -> realign_b_im/1
  a_im/1 -> realign_a_im/1
  carryinsel/1 -> DSP48E/7
  carryin/1 -> DSP48E/6
  alumode/1 -> DSP48E/5
  opmode/1 -> DSP48E/4
  Reinterpret_B/1 -> DSP48E/2
  Reinterpret_A/1 -> DSP48E/1
  b_re/1 -> realign_b_re/1
  a_re/1 -> realign_a_re/1
  realign_a_re/1 -> reinterp_a_re/1
  realign_a_im/1 -> reinterp_a_im/1
  realign_b_re/1 -> reinterp_b_re/1
  realign_b_im/1 -> reinterp_b_im/1

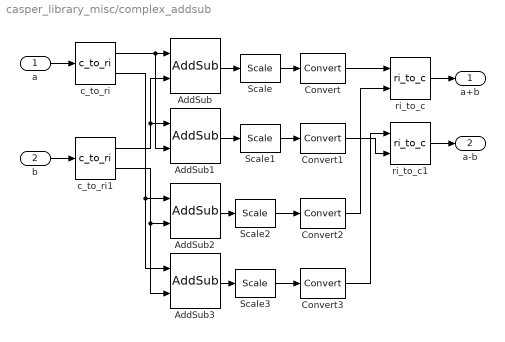
== system casper_library_misc/complex_addsub ==
  a : Inport
  b : Inport  Port=2
  AddSub : xbsIndex_r4/AddSub  mode=Addition  use_carryin=off  use_carryout=off  en=off  latency=add_latency  precision=Full  arith_type=Unsigned  n_bits=8  bin_pt=2  quantization=Truncate  overflow=Wrap  use_behavioral_HDL=on  hw_selection=Fabric  pipelined=off  use_rpm=on  dbl_ovrd=off  block_type=addsub
      settings: xl_area=[0, 0, 0, 0, 0, 0, 0]  block_version=9.1.01
  AddSub1 : xbsIndex_r4/AddSub  mode=Subtraction  use_carryin=off  use_carryout=off  en=off  latency=add_latency  precision=Full  arith_type=Unsigned  n_bits=8  bin_pt=2  quantization=Truncate  overflow=Wrap  use_behavioral_HDL=on  hw_selection=Fabric  pipelined=off  use_rpm=on  dbl_ovrd=off  block_type=addsub
      settings: xl_area=[0, 0, 0, 0, 0, 0, 0]  block_version=9.1.01
  AddSub2 : xbsIndex_r4/AddSub  mode=Subtraction  use_carryin=off  use_carryout=off  en=off  latency=add_latency  precision=Full  arith_type=Unsigned  n_bits=8  bin_pt=2  quantization=Truncate  overflow=Wrap  use_behavioral_HDL=on  hw_selection=Fabric  pipelined=off  use_rpm=on  dbl_ovrd=off  block_type=addsub
      settings: xl_area=[0, 0, 0, 0, 0, 0, 0]  block_version=9.1.01
  AddSub3 : xbsIndex_r4/AddSub  mode=Addition  use_carryin=off  use_carryout=off  en=off  latency=add_latency  precision=Full  arith_type=Unsigned  n_bits=8  bin_pt=2  quantization=Truncate  overflow=Wrap  use_behavioral_HDL=on  hw_selection=Fabric  pipelined=off  use_rpm=on  dbl_ovrd=off  block_type=addsub
      settings: xl_area=[0, 0, 0, 0, 0, 0, 0]  block_version=9.1.01
  Convert{,1..3} (4 alike) : xbsIndex_r4/Convert  gui_display_data_type=Fixed-point  arith_type="Signed  (2's comp)"  n_bits=BitWidth  bin_pt=BitWidth - 1  float_type=Single  exp_bits=8  fraction_bits=24  quantization="Round  (unbiased: Even Values)"  overflow=Wrap  en=off  latency=add_latency  pipeline=off  dbl_ovrd=off  block_type=convert
      settings: xl_area=[0, 0, 0, 0, 0, 0, 0]
  Scale{,1..3} (4 alike) : xbsIndex_r4/Scale  scale_factor=-1  dbl_ovrd=off  block_type=scale
  c_to_ri : $bdroot/c_to_ri  n_bits=BitWidth  bin_pt=BitWidth-1
      settings: AttributesFormatString=18_17 r/i
  c_to_ri1 : $bdroot/c_to_ri  n_bits=BitWidth  bin_pt=BitWidth-1
      settings: AttributesFormatString=18_17 r/i
  ri_to_c : $bdroot/ri_to_c
  ri_to_c1 : $bdroot/ri_to_c
  a+b : Outport  VectorParamsAs1DForOutWhenUnconnected=off
  a-b : Outport  Port=2  VectorParamsAs1DForOutWhenUnconnected=off
  wires:
  Scale3/1 -> Convert3/1
  Scale2/1 -> Convert2/1
  Scale1/1 -> Convert1/1
  Scale/1 -> Convert/1
  b/1 -> c_to_ri1/1
  ri_to_c1/1 -> a-b/1
  ri_to_c/1 -> a+b/1
  a/1 -> c_to_ri/1
  Convert2/1 -> ri_to_c/2
  Convert/1 -> ri_to_c/1
  c_to_ri1/2 -> AddSub3/2, AddSub2/2
  c_to_ri1/1 -> AddSub/2, AddSub1/1
  c_to_ri/2 -> AddSub3/1, AddSub2/1
  c_to_ri/1 -> AddSub/1, AddSub1/2
  AddSub3/1 -> Scale3/1
  AddSub2/1 -> Scale2/1
  AddSub1/1 -> Scale1/1
  AddSub/1 -> Scale/1
  Convert1/1 -> ri_to_c1/2
  Convert3/1 -> ri_to_c1/1

== system casper_library_misc/complex_conj ==
